simulink model "TB11_R2_FaultMod_SW"  (R2025a)
settings: Solver=FixedStepDiscrete  StartTime=0  StopTime=TB.t_end  FixedStep=TB.dt  RelTol=1e-3
InitFcn:
  | % 모델과 같은 폴더의 초기화 스크립트를 실행해 P(설계 파라미터)와 TB(시험 조건)를 만든다.
  | run(fullfile(fileparts(get_param(bdroot, 'FileName')), 'TB11_init.m'));
values from neighbouring files (symbols this model uses):
  TB = struct()    [TB11_init.m]    (also in run_TB11.m = evalin('base', 'TB'))
libraries: fl_lib x68, nesl_utility x29
(part 2 of 2)

== system TB11_R2_FaultMod_SW/StageB_Regulator/DAB_Primary/P4_leg2_low ==
  note: 스위치 셀: 이상 스위치(R_on, G_off) + 역병렬 바디 다이오드(Vf, R_d) + 출력용량 C_oss
      | 게이트: 전역 태그 "gD_P4" (> 0.5 이면 도통)
  C_oss : fl_lib/Electrical/Electrical Elements/Capacitor  c=Coss F  r=1e-6 Ohm  g=0 1/Ohm  i_specify=off  i_priority=None  i=0 A  i_nominal_specify=off  i_nominal_value=1  i_nominal_unit=A  v_specify=off  v_priority=None  v=0 V  v_nominal_specify=off  v_nominal_value=1  v_nominal_unit=V  vc_specify=off  vc_priority=High  vc=0 V  vc_nominal_specify=off  vc_nominal_value=1  vc_nominal_unit=V
  D_body : fl_lib/Electrical/Electrical Elements/Diode  Vf=Vf V  Ron=Rd Ohm  Goff=Goffd 1/Ohm  i_specify=off  i_priority=None  i=0 A  i_nominal_specify=off  i_nominal_value=1  i_nominal_unit=A  v_specify=off  v_priority=None  v=0 V  v_nominal_specify=off  v_nominal_value=1  v_nominal_unit=V
  Gate_PS : nesl_utility/Simulink-PS Converter  PhysicalDomain=network_engine_domain  SubClassName=ps_input  LeftPortType=input  RightPortType=output  PseudoPeriodic=off  Frequencies=[]  NoiseDistribution=none  NoiseParameters=[]  Unit=1  AffineConversion=off  FilteringAndDerivatives=zero  SimscapeFilterOrder=1  InputFilterTimeConstant=0.001  UdotUserProvided=0
  SW : fl_lib/Electrical/Electrical Elements/Switch  R_closed=Ron Ohm  G_open=Goff 1/Ohm  Threshold=0.5  i_specify=off  i_priority=None  i=0 A  i_nominal_specify=off  i_nominal_value=1  i_nominal_unit=A  v_specify=off  v_priority=None  v=0 V  v_nominal_specify=off  v_nominal_value=1  v_nominal_unit=V
  D : PMIOPort  Side=Left
  S : PMIOPort  Port=2  Side=Right
  wires:
  [gD_P4] -> Gate_PS/1
  connections:
  Gate_PS/RConn1 -- SW/RConn1
  SW/LConn1 -- D/RConn1 -- D_body/RConn1 -- C_oss/LConn1
  SW/RConn2 -- D_body/LConn1 -- S/RConn1 -- C_oss/RConn1

== system TB11_R2_FaultMod_SW/StageB_Regulator/DAB_Secondary/S1_leg1_high ==
  note: 스위치 셀: 이상 스위치(R_on, G_off) + 역병렬 바디 다이오드(Vf, R_d) + 출력용량 C_oss
      | 게이트: 전역 태그 "gD_S1" (> 0.5 이면 도통)
  C_oss : fl_lib/Electrical/Electrical Elements/Capacitor  c=Coss F  r=1e-6 Ohm  g=0 1/Ohm  i_specify=off  i_priority=None  i=0 A  i_nominal_specify=off  i_nominal_value=1  i_nominal_unit=A  v_specify=off  v_priority=None  v=0 V  v_nominal_specify=off  v_nominal_value=1  v_nominal_unit=V  vc_specify=off  vc_priority=High  vc=0 V  vc_nominal_specify=off  vc_nominal_value=1  vc_nominal_unit=V
  D_body : fl_lib/Electrical/Electrical Elements/Diode  Vf=Vf V  Ron=Rd Ohm  Goff=Goffd 1/Ohm  i_specify=off  i_priority=None  i=0 A  i_nominal_specify=off  i_nominal_value=1  i_nominal_unit=A  v_specify=off  v_priority=None  v=0 V  v_nominal_specify=off  v_nominal_value=1  v_nominal_unit=V
  Gate_PS : nesl_utility/Simulink-PS Converter  PhysicalDomain=network_engine_domain  SubClassName=ps_input  LeftPortType=input  RightPortType=output  PseudoPeriodic=off  Frequencies=[]  NoiseDistribution=none  NoiseParameters=[]  Unit=1  AffineConversion=off  FilteringAndDerivatives=zero  SimscapeFilterOrder=1  InputFilterTimeConstant=0.001  UdotUserProvided=0
  SW : fl_lib/Electrical/Electrical Elements/Switch  R_closed=Ron Ohm  G_open=Goff 1/Ohm  Threshold=0.5  i_specify=off  i_priority=None  i=0 A  i_nominal_specify=off  i_nominal_value=1  i_nominal_unit=A  v_specify=off  v_priority=None  v=0 V  v_nominal_specify=off  v_nominal_value=1  v_nominal_unit=V
  D : PMIOPort  Side=Left
  S : PMIOPort  Port=2  Side=Right
  wires:
  [gD_S1] -> Gate_PS/1
  connections:
  Gate_PS/RConn1 -- SW/RConn1
  SW/LConn1 -- D/RConn1 -- D_body/RConn1 -- C_oss/LConn1
  SW/RConn2 -- D_body/LConn1 -- S/RConn1 -- C_oss/RConn1

== system TB11_R2_FaultMod_SW/StageB_Regulator/DAB_Secondary/S2_leg1_low ==
  note: 스위치 셀: 이상 스위치(R_on, G_off) + 역병렬 바디 다이오드(Vf, R_d) + 출력용량 C_oss
      | 게이트: 전역 태그 "gD_S2" (> 0.5 이면 도통)
  C_oss : fl_lib/Electrical/Electrical Elements/Capacitor  c=Coss F  r=1e-6 Ohm  g=0 1/Ohm  i_specify=off  i_priority=None  i=0 A  i_nominal_specify=off  i_nominal_value=1  i_nominal_unit=A  v_specify=off  v_priority=None  v=0 V  v_nominal_specify=off  v_nominal_value=1  v_nominal_unit=V  vc_specify=off  vc_priority=High  vc=0 V  vc_nominal_specify=off  vc_nominal_value=1  vc_nominal_unit=V
  D_body : fl_lib/Electrical/Electrical Elements/Diode  Vf=Vf V  Ron=Rd Ohm  Goff=Goffd 1/Ohm  i_specify=off  i_priority=None  i=0 A  i_nominal_specify=off  i_nominal_value=1  i_nominal_unit=A  v_specify=off  v_priority=None  v=0 V  v_nominal_specify=off  v_nominal_value=1  v_nominal_unit=V
  Gate_PS : nesl_utility/Simulink-PS Converter  PhysicalDomain=network_engine_domain  SubClassName=ps_input  LeftPortType=input  RightPortType=output  PseudoPeriodic=off  Frequencies=[]  NoiseDistribution=none  NoiseParameters=[]  Unit=1  AffineConversion=off  FilteringAndDerivatives=zero  SimscapeFilterOrder=1  InputFilterTimeConstant=0.001  UdotUserProvided=0
  SW : fl_lib/Electrical/Electrical Elements/Switch  R_closed=Ron Ohm  G_open=Goff 1/Ohm  Threshold=0.5  i_specify=off  i_priority=None  i=0 A  i_nominal_specify=off  i_nominal_value=1  i_nominal_unit=A  v_specify=off  v_priority=None  v=0 V  v_nominal_specify=off  v_nominal_value=1  v_nominal_unit=V
  D : PMIOPort  Side=Left
  S : PMIOPort  Port=2  Side=Right
  wires:
  [gD_S2] -> Gate_PS/1
  connections:
  Gate_PS/RConn1 -- SW/RConn1
  SW/LConn1 -- D/RConn1 -- D_body/RConn1 -- C_oss/LConn1
  SW/RConn2 -- D_body/LConn1 -- S/RConn1 -- C_oss/RConn1

== system TB11_R2_FaultMod_SW/StageB_Regulator/DAB_Secondary/S3_leg2_high ==
  note: 스위치 셀: 이상 스위치(R_on, G_off) + 역병렬 바디 다이오드(Vf, R_d) + 출력용량 C_oss
      | 게이트: 전역 태그 "gD_S3" (> 0.5 이면 도통)
  C_oss : fl_lib/Electrical/Electrical Elements/Capacitor  c=Coss F  r=1e-6 Ohm  g=0 1/Ohm  i_specify=off  i_priority=None  i=0 A  i_nominal_specify=off  i_nominal_value=1  i_nominal_unit=A  v_specify=off  v_priority=None  v=0 V  v_nominal_specify=off  v_nominal_value=1  v_nominal_unit=V  vc_specify=off  vc_priority=High  vc=0 V  vc_nominal_specify=off  vc_nominal_value=1  vc_nominal_unit=V
  D_body : fl_lib/Electrical/Electrical Elements/Diode  Vf=Vf V  Ron=Rd Ohm  Goff=Goffd 1/Ohm  i_specify=off  i_priority=None  i=0 A  i_nominal_specify=off  i_nominal_value=1  i_nominal_unit=A  v_specify=off  v_priority=None  v=0 V  v_nominal_specify=off  v_nominal_value=1  v_nominal_unit=V
  Gate_PS : nesl_utility/Simulink-PS Converter  PhysicalDomain=network_engine_domain  SubClassName=ps_input  LeftPortType=input  RightPortType=output  PseudoPeriodic=off  Frequencies=[]  NoiseDistribution=none  NoiseParameters=[]  Unit=1  AffineConversion=off  FilteringAndDerivatives=zero  SimscapeFilterOrder=1  InputFilterTimeConstant=0.001  UdotUserProvided=0
  SW : fl_lib/Electrical/Electrical Elements/Switch  R_closed=Ron Ohm  G_open=Goff 1/Ohm  Threshold=0.5  i_specify=off  i_priority=None  i=0 A  i_nominal_specify=off  i_nominal_value=1  i_nominal_unit=A  v_specify=off  v_priority=None  v=0 V  v_nominal_specify=off  v_nominal_value=1  v_nominal_unit=V
  D : PMIOPort  Side=Left
  S : PMIOPort  Port=2  Side=Right
  wires:
  [gD_S3] -> Gate_PS/1
  connections:
  Gate_PS/RConn1 -- SW/RConn1
  SW/LConn1 -- D/RConn1 -- D_body/RConn1 -- C_oss/LConn1
  SW/RConn2 -- D_body/LConn1 -- S/RConn1 -- C_oss/RConn1

== system TB11_R2_FaultMod_SW/StageB_Regulator/DAB_Secondary/S4_leg2_low ==
  note: 스위치 셀: 이상 스위치(R_on, G_off) + 역병렬 바디 다이오드(Vf, R_d) + 출력용량 C_oss
      | 게이트: 전역 태그 "gD_S4" (> 0.5 이면 도통)
  C_oss : fl_lib/Electrical/Electrical Elements/Capacitor  c=Coss F  r=1e-6 Ohm  g=0 1/Ohm  i_specify=off  i_priority=None  i=0 A  i_nominal_specify=off  i_nominal_value=1  i_nominal_unit=A  v_specify=off  v_priority=None  v=0 V  v_nominal_specify=off  v_nominal_value=1  v_nominal_unit=V  vc_specify=off  vc_priority=High  vc=0 V  vc_nominal_specify=off  vc_nominal_value=1  vc_nominal_unit=V
  D_body : fl_lib/Electrical/Electrical Elements/Diode  Vf=Vf V  Ron=Rd Ohm  Goff=Goffd 1/Ohm  i_specify=off  i_priority=None  i=0 A  i_nominal_specify=off  i_nominal_value=1  i_nominal_unit=A  v_specify=off  v_priority=None  v=0 V  v_nominal_specify=off  v_nominal_value=1  v_nominal_unit=V
  Gate_PS : nesl_utility/Simulink-PS Converter  PhysicalDomain=network_engine_domain  SubClassName=ps_input  LeftPortType=input  RightPortType=output  PseudoPeriodic=off  Frequencies=[]  NoiseDistribution=none  NoiseParameters=[]  Unit=1  AffineConversion=off  FilteringAndDerivatives=zero  SimscapeFilterOrder=1  InputFilterTimeConstant=0.001  UdotUserProvided=0
  SW : fl_lib/Electrical/Electrical Elements/Switch  R_closed=Ron Ohm  G_open=Goff 1/Ohm  Threshold=0.5  i_specify=off  i_priority=None  i=0 A  i_nominal_specify=off  i_nominal_value=1  i_nominal_unit=A  v_specify=off  v_priority=None  v=0 V  v_nominal_specify=off  v_nominal_value=1  v_nominal_unit=V
  D : PMIOPort  Side=Left
  S : PMIOPort  Port=2  Side=Right
  wires:
  [gD_S4] -> Gate_PS/1
  connections:
  Gate_PS/RConn1 -- SW/RConn1
  SW/LConn1 -- D/RConn1 -- D_body/RConn1 -- C_oss/LConn1
  SW/RConn2 -- D_body/LConn1 -- S/RConn1 -- C_oss/RConn1

== system TB11_R2_FaultMod_SW/StageB_Regulator/HBridge/QA_high ==
  note: 스위치 셀: 이상 스위치(R_on, G_off) + 역병렬 바디 다이오드(Vf, R_d) + 출력용량 C_oss
      | 게이트: 전역 태그 "gB_AH" (> 0.5 이면 도통)
  C_oss : fl_lib/Electrical/Electrical Elements/Capacitor  c=Coss F  r=1e-6 Ohm  g=0 1/Ohm  i_specify=off  i_priority=None  i=0 A  i_nominal_specify=off  i_nominal_value=1  i_nominal_unit=A  v_specify=off  v_priority=None  v=0 V  v_nominal_specify=off  v_nominal_value=1  v_nominal_unit=V  vc_specify=off  vc_priority=High  vc=0 V  vc_nominal_specify=off  vc_nominal_value=1  vc_nominal_unit=V
  D_body : fl_lib/Electrical/Electrical Elements/Diode  Vf=Vf V  Ron=Rd Ohm  Goff=Goffd 1/Ohm  i_specify=off  i_priority=None  i=0 A  i_nominal_specify=off  i_nominal_value=1  i_nominal_unit=A  v_specify=off  v_priority=None  v=0 V  v_nominal_specify=off  v_nominal_value=1  v_nominal_unit=V
  Gate_PS : nesl_utility/Simulink-PS Converter  PhysicalDomain=network_engine_domain  SubClassName=ps_input  LeftPortType=input  RightPortType=output  PseudoPeriodic=off  Frequencies=[]  NoiseDistribution=none  NoiseParameters=[]  Unit=1  AffineConversion=off  FilteringAndDerivatives=zero  SimscapeFilterOrder=1  InputFilterTimeConstant=0.001  UdotUserProvided=0
  SW : fl_lib/Electrical/Electrical Elements/Switch  R_closed=Ron Ohm  G_open=Goff 1/Ohm  Threshold=0.5  i_specify=off  i_priority=None  i=0 A  i_nominal_specify=off  i_nominal_value=1  i_nominal_unit=A  v_specify=off  v_priority=None  v=0 V  v_nominal_specify=off  v_nominal_value=1  v_nominal_unit=V
  D : PMIOPort  Side=Left
  S : PMIOPort  Port=2  Side=Right
  wires:
  [gB_AH] -> Gate_PS/1
  connections:
  Gate_PS/RConn1 -- SW/RConn1
  SW/LConn1 -- D/RConn1 -- D_body/RConn1 -- C_oss/LConn1
  SW/RConn2 -- D_body/LConn1 -- S/RConn1 -- C_oss/RConn1

== system TB11_R2_FaultMod_SW/StageB_Regulator/HBridge/QA_low ==
  note: 스위치 셀: 이상 스위치(R_on, G_off) + 역병렬 바디 다이오드(Vf, R_d) + 출력용량 C_oss
      | 게이트: 전역 태그 "gB_AL" (> 0.5 이면 도통)
  C_oss : fl_lib/Electrical/Electrical Elements/Capacitor  c=Coss F  r=1e-6 Ohm  g=0 1/Ohm  i_specify=off  i_priority=None  i=0 A  i_nominal_specify=off  i_nominal_value=1  i_nominal_unit=A  v_specify=off  v_priority=None  v=0 V  v_nominal_specify=off  v_nominal_value=1  v_nominal_unit=V  vc_specify=off  vc_priority=High  vc=0 V  vc_nominal_specify=off  vc_nominal_value=1  vc_nominal_unit=V
  D_body : fl_lib/Electrical/Electrical Elements/Diode  Vf=Vf V  Ron=Rd Ohm  Goff=Goffd 1/Ohm  i_specify=off  i_priority=None  i=0 A  i_nominal_specify=off  i_nominal_value=1  i_nominal_unit=A  v_specify=off  v_priority=None  v=0 V  v_nominal_specify=off  v_nominal_value=1  v_nominal_unit=V
  Gate_PS : nesl_utility/Simulink-PS Converter  PhysicalDomain=network_engine_domain  SubClassName=ps_input  LeftPortType=input  RightPortType=output  PseudoPeriodic=off  Frequencies=[]  NoiseDistribution=none  NoiseParameters=[]  Unit=1  AffineConversion=off  FilteringAndDerivatives=zero  SimscapeFilterOrder=1  InputFilterTimeConstant=0.001  UdotUserProvided=0
  SW : fl_lib/Electrical/Electrical Elements/Switch  R_closed=Ron Ohm  G_open=Goff 1/Ohm  Threshold=0.5  i_specify=off  i_priority=None  i=0 A  i_nominal_specify=off  i_nominal_value=1  i_nominal_unit=A  v_specify=off  v_priority=None  v=0 V  v_nominal_specify=off  v_nominal_value=1  v_nominal_unit=V
  D : PMIOPort  Side=Left
  S : PMIOPort  Port=2  Side=Right
  wires:
  [gB_AL] -> Gate_PS/1
  connections:
  Gate_PS/RConn1 -- SW/RConn1
  SW/LConn1 -- D/RConn1 -- D_body/RConn1 -- C_oss/LConn1
  SW/RConn2 -- D_body/LConn1 -- S/RConn1 -- C_oss/RConn1

== system TB11_R2_FaultMod_SW/StageB_Regulator/HBridge/QB_high ==
  note: 스위치 셀: 이상 스위치(R_on, G_off) + 역병렬 바디 다이오드(Vf, R_d) + 출력용량 C_oss
      | 게이트: 전역 태그 "gB_BH" (> 0.5 이면 도통)
  C_oss : fl_lib/Electrical/Electrical Elements/Capacitor  c=Coss F  r=1e-6 Ohm  g=0 1/Ohm  i_specify=off  i_priority=None  i=0 A  i_nominal_specify=off  i_nominal_value=1  i_nominal_unit=A  v_specify=off  v_priority=None  v=0 V  v_nominal_specify=off  v_nominal_value=1  v_nominal_unit=V  vc_specify=off  vc_priority=High  vc=0 V  vc_nominal_specify=off  vc_nominal_value=1  vc_nominal_unit=V
  D_body : fl_lib/Electrical/Electrical Elements/Diode  Vf=Vf V  Ron=Rd Ohm  Goff=Goffd 1/Ohm  i_specify=off  i_priority=None  i=0 A  i_nominal_specify=off  i_nominal_value=1  i_nominal_unit=A  v_specify=off  v_priority=None  v=0 V  v_nominal_specify=off  v_nominal_value=1  v_nominal_unit=V
  Gate_PS : nesl_utility/Simulink-PS Converter  PhysicalDomain=network_engine_domain  SubClassName=ps_input  LeftPortType=input  RightPortType=output  PseudoPeriodic=off  Frequencies=[]  NoiseDistribution=none  NoiseParameters=[]  Unit=1  AffineConversion=off  FilteringAndDerivatives=zero  SimscapeFilterOrder=1  InputFilterTimeConstant=0.001  UdotUserProvided=0
  SW : fl_lib/Electrical/Electrical Elements/Switch  R_closed=Ron Ohm  G_open=Goff 1/Ohm  Threshold=0.5  i_specify=off  i_priority=None  i=0 A  i_nominal_specify=off  i_nominal_value=1  i_nominal_unit=A  v_specify=off  v_priority=None  v=0 V  v_nominal_specify=off  v_nominal_value=1  v_nominal_unit=V
  D : PMIOPort  Side=Left
  S : PMIOPort  Port=2  Side=Right
  wires:
  [gB_BH] -> Gate_PS/1
  connections:
  Gate_PS/RConn1 -- SW/RConn1
  SW/LConn1 -- D/RConn1 -- D_body/RConn1 -- C_oss/LConn1
  SW/RConn2 -- D_body/LConn1 -- S/RConn1 -- C_oss/RConn1

== system TB11_R2_FaultMod_SW/StageB_Regulator/HBridge/QB_low ==
  note: 스위치 셀: 이상 스위치(R_on, G_off) + 역병렬 바디 다이오드(Vf, R_d) + 출력용량 C_oss
      | 게이트: 전역 태그 "gB_BL" (> 0.5 이면 도통)
  C_oss : fl_lib/Electrical/Electrical Elements/Capacitor  c=Coss F  r=1e-6 Ohm  g=0 1/Ohm  i_specify=off  i_priority=None  i=0 A  i_nominal_specify=off  i_nominal_value=1  i_nominal_unit=A  v_specify=off  v_priority=None  v=0 V  v_nominal_specify=off  v_nominal_value=1  v_nominal_unit=V  vc_specify=off  vc_priority=High  vc=0 V  vc_nominal_specify=off  vc_nominal_value=1  vc_nominal_unit=V
  D_body : fl_lib/Electrical/Electrical Elements/Diode  Vf=Vf V  Ron=Rd Ohm  Goff=Goffd 1/Ohm  i_specify=off  i_priority=None  i=0 A  i_nominal_specify=off  i_nominal_value=1  i_nominal_unit=A  v_specify=off  v_priority=None  v=0 V  v_nominal_specify=off  v_nominal_value=1  v_nominal_unit=V
  Gate_PS : nesl_utility/Simulink-PS Converter  PhysicalDomain=network_engine_domain  SubClassName=ps_input  LeftPortType=input  RightPortType=output  PseudoPeriodic=off  Frequencies=[]  NoiseDistribution=none  NoiseParameters=[]  Unit=1  AffineConversion=off  FilteringAndDerivatives=zero  SimscapeFilterOrder=1  InputFilterTimeConstant=0.001  UdotUserProvided=0
  SW : fl_lib/Electrical/Electrical Elements/Switch  R_closed=Ron Ohm  G_open=Goff 1/Ohm  Threshold=0.5  i_specify=off  i_priority=None  i=0 A  i_nominal_specify=off  i_nominal_value=1  i_nominal_unit=A  v_specify=off  v_priority=None  v=0 V  v_nominal_specify=off  v_nominal_value=1  v_nominal_unit=V
  D : PMIOPort  Side=Left
  S : PMIOPort  Port=2  Side=Right
  wires:
  [gB_BL] -> Gate_PS/1
  connections:
  Gate_PS/RConn1 -- SW/RConn1
  SW/LConn1 -- D/RConn1 -- D_body/RConn1 -- C_oss/LConn1
  SW/RConn2 -- D_body/LConn1 -- S/RConn1 -- C_oss/RConn1

== matlab function TB11_R2_FaultMod_SW/Controller_StageB/R2_Supervisor ==
  data: t input; s output; y input; fl input; prm input; smp input
function s = prism_r2_sup_sampler(t, y, fl, prm, smp)
%#codegen
%PRISM_R2_SUP_SAMPLER  R2 보호 상태기계 표본화 실행기(TB09, MATLAB Function 블록의 진입 함수).
%
%   5 µs마다(제어기와 같은 표본 시점, 제어기보다 먼저) ctrl/prism_r2_supervisor.m을 한 번 계산하고 그 밖에는 직전 출력을 유지한다.
%   입력  t 시각, y [i_p v_s v_bus i_h v_link], fl [게이트 구동기 고장 신호, 비교기 차단 래치](한 간격 지연),
%         prm 상태기계 파라미터(TB.sup_prm), smp [dt Np]
%   출력  s 상태기계 지령 12개(prism_r2_supervisor.m 참조)

persistent sh
if isempty(sh)
    sh = zeros(12, 1);
end
k = round(t/smp(1));
if mod(k, round(smp(2))) == 0
    sh = prism_r2_supervisor(t, y, fl, prm);
end
s = sh;
end

function s = prism_r2_supervisor(t, y, fl, prm)
%#codegen
%PRISM_R2_SUPERVISOR  R2 창 조정 모듈의 측정 기반 보호 상태기계(TB09, 검증 코드 E17 r2_run의 상태기계와 같은 논리).
%
%  5 µs마다(호출 측 표본기) 측정값과 고장 신호로 운전 상태를 정하고, 제어기·게이트·바이패스·제동 저항·부하 분리 명령을 낸다.
%  상태 번호
%    0 바이패스          바이패스 닫힘, H-브리지·DAB 정지(버스 = V_A)
%    1 준비(PREP)        바이패스 + H-브리지(영벡터 또는 전류 조향: 바이패스 전류 → 0)
%    2 열림 대기         바이패스 열림, H-브리지 영벡터(또는 조향) → t_wait 뒤 제어 시작
%    3 창 조정           채택 제어기(기준 V_A → V_W 램프 뒤 V_W)
%    4 끔 램프 / 5 끔 유지(기준 = V_A 추정, |v_s| ≤ 2 V가 50 µs 이어지면) / 6 영벡터(또는 직렬전압 조향) → 바이패스
%    7 DAB 고장 유지     H-브리지는 계속 조정, DAB 정지, 링크 제동 저항으로 링크 ≤ 110 V, 400 V 부하 분리 대기
%    8 DAB 고장 램프     기준 → V_A(1 ms) → V_A 추정 추종, |v_s| ≤ 2 V가 50 µs 이어지면 → 6 → 강등
%    9 H-브리지 고장 유지  H-브리지 꺼짐(다이오드 정류), DAB 보조 루프가 링크전압으로 버스를 V_W에 붙잡음 + 제동 저항
%   10 링크 붕괴         링크 기준을 20 V/ms로 0 V까지 → 직렬전압이 다이오드 전압까지 줄어듦.
%                        링크 ≤ VL_SOFT, 또는 정체(기준 0 도달 뒤 T_STALL 동안 DV_STALL도 안 내려가고 링크 ≤ VL_STALL), 또는 T_COL_MAX → 11
%   11 소프트 바이패스   바이패스 저항을 10 Ω에서 로그 램프로 낮추되(제한 없으면 T_SOFT에 3.3 mΩ), 경로전류가 투입 시작값 + DI_SOFT를
%                        넘으면 표본마다 K_UP배로 되올린다(경로전류 조절). 3.3 mΩ에 이르거나 T_SOFT_MAX가 지나면 → 12
%   12 강등              바이패스 닫힘, Stage B 정지(버스 = V_A)
%   13 이중 고장         DAB 고장 중 H-브리지 차단: Stage A 협조 정지가 필요(이 모델 밖)
%
%  (2026-10-24 TB09 1차 결과로 추가: 회로에서는 링크 붕괴가 3.5–22 V에서 멈췄고, 남은 직렬전압을 로그 램프로 닫자 경로전류가
%   177 A까지 올랐다. 그래서 정체 감지와 경로전류 조절을 넣었다. 같은 논리를 검증 코드 E17에도 넣었다.)
%
%  (2026-10-24 TB10, 검증 코드 E20: prm이 60개면 다음을 켠다. 56개(TB09)면 이전과 같다.)
%   prm(57) 전압비 정합 유지(1): H-브리지 강등 유지(9)의 링크 기준 = (V_A − (R + R_h)i_p − 2V_D)/(n + 1), 제동 저항은 기준 추종
%   prm(58) 일시 감발(1): H-브리지 고장이면 V_A와 무관하게 400 V 부하 출력을 줄이고, V_A ≤ 상한이면 강등 T_RESTORE 뒤 되돌림
%   prm(59) 소프트 투입 시간 상한이면 주 스위치를 닫지 않고 이중 고장(13)으로
%   prm(60) T_RESTORE [s]
%   DAB 변조(EPS)와 첨두 상한은 게이트 쪽 ctrl/prism_dab_eps_map.m이 맡는다(상태 9–11, DAB 모드 1).
%
%  입력  t    시각 [s]
%        y    측정 [i_p v_s v_bus i_h v_link]
%        fl   [게이트 구동기 고장 신호(H-브리지 개방), 하드웨어 비교기 차단 래치]
%        prm  파라미터 벡터(TB09_init.m의 TB.sup_prm, 번호는 아래 코드 주석)
%  출력  s = [V_ref; 재초기화; 브리지 모드(0 제어 PWM, 1 영벡터, 2 차단, 3 조향 PWM); 조향 변조율;
%             DAB 모드(0 제어기, 1 보조 지령, 2 정지); 보조 링크전류 지령; 바이패스 소프트 저항 [Ω]; 바이패스 주 스위치(1/0);
%             제동 저항 게이트(1/0); 400 V 부하 분리(1/0); 상태 번호; 고장 검출(0 없음, 1 구동기, 2 비교기, 3 링크 창, 4 버스 창)]

persistent st t_st t_det det shed_cmd shed sw_since vb_since rv0 rv1 rt1 rtype qb amode vl0 t0 tsoft0 Rs main brk mst gsince ip_s0 stall_t stall_v ...
           curt_only restored
VW = prm(1); upper = prm(2); H = prm(3); R = prm(4); Rh = prm(5); Cs = prm(6); Lh = prm(7); itau = prm(8);
Clink = prm(9); VD = prm(10); t_ev = prm(11); ev = prm(12); pol = prm(13); prep = prm(14); cls = prm(15);
t_prep = prm(16); t_wait = prm(17); RAMP = prm(18); HOLD = prm(19); ZERO = prm(20); t_shed = prm(21);
RATE = prm(22); VL_SOFT = prm(23); T_SOFT = prm(24); R_SOFT0 = prm(25); R_ON = prm(26); T_COL_MAX = prm(27);
VL_LO = prm(28); VL_HI = prm(29); T_SW = prm(30); VB_SW = prm(31); T_VB = prm(32);
KP_B = prm(33); KI_B = prm(34); QB_MAX = prm(35); W_L = prm(36); TAU_ST = prm(37); R_OPEN = prm(38);
P_r = prm(39); link_max = prm(40); turns = prm(41); phmax = prm(42); fs = prm(43); Ldab = prm(44); vbat = prm(45);
st0 = prm(46); Ts = prm(47); VS_GATE = prm(48); T_GATE = prm(49); T_GATE_MAX = prm(50);
VL_STALL = prm(51); T_STALL = prm(52); DV_STALL = prm(53); DI_SOFT = prm(54); K_UP = prm(55); T_SOFT_MAX = prm(56);
K_DN = (R_SOFT0/R_ON)^(Ts/T_SOFT);                    % 제한에 안 걸리면 10 Ω → 3.3 mΩ를 T_SOFT에 지나는 표본당 비율
HOLD_MATCH = 0; CURTAIL = 0; SOFT_FAIL = 0; T_RESTORE = 0.5e-3;
if numel(prm) >= 60
    HOLD_MATCH = prm(57); CURTAIL = prm(58); SOFT_FAIL = prm(59); T_RESTORE = prm(60);
end

ip = y(1); vs = y(2); vb = y(3); ih = y(4); vl = y(5);
if isempty(st)
    st = st0; t_st = 0; t_det = -1; det = 0; shed_cmd = -1; shed = 0; sw_since = -1; vb_since = -1;
    rv0 = VW; rv1 = VW; rt1 = 0; rtype = 0; qb = 0; amode = 0; vl0 = 100; t0 = 0; tsoft0 = 0;
    if st0 == 3, Rs = R_OPEN; main = 0; else, Rs = R_OPEN; main = 1; end
    brk = 0; mst = 0; gsince = -1; ip_s0 = 0; stall_t = -1; stall_v = 0; curt_only = 0; restored = 0;
end
va_m = vbat/2 - R*ip;                                  % V_A 추정(배터리 전압 센서 − 경로 강하)
gwin = (st == 5 && t - t_st >= HOLD - 1e-12) || (st == 8 && t - t_st >= RAMP + HOLD - 1e-12);
if gwin && abs(vs) <= VS_GATE                          % 영벡터 진입 조건: 최소 유지 뒤 |v_s| ≤ 2 V가 50 µs 이어짐
    if gsince < 0, gsince = t; end
else
    gsince = -1;
end
gate_ok = gsince >= 0 && t - gsince >= T_GATE - 1e-12;
bridge_dead = fl(1) > 0.5 || fl(2) > 0.5;
% ---- 고장 검출 --------------------------------------------------------------------------------
if t_det < 0
    if fl(1) > 0.5, t_det = t; det = 1; end
    if fl(2) > 0.5, t_det = t; det = 2; end
    if t_det < 0 && (st == 3 || st == 4 || st == 5)
        if vl < VL_LO || vl > VL_HI
            if sw_since < 0, sw_since = t; end
            if t - sw_since >= T_SW - 1e-12, t_det = t; det = 3; end
        else
            sw_since = -1;
        end
        if abs(vb - vref_at(t, rtype, rv0, rv1, rt1, RAMP, VW, va_m)) > VB_SW
            if vb_since < 0, vb_since = t; end
            if t - vb_since >= T_VB - 1e-12, t_det = t; det = 4; end
        else
            vb_since = -1;
        end
    end
elseif fl(2) > 0.5 && det == 3 && st ~= 13 && st ~= 12 && st >= 6 && st <= 8
    st = 13; t_st = t;                                  % DAB 고장 강등 중 하드웨어 차단 → 이중 고장
end
sw_states = (st >= 1 && st <= 8);
hb_det = det == 1 || det == 2 || det == 4;
if t_det >= 0 && shed_cmd < 0 && st ~= 0 && (va_m > upper - 2 || (CURTAIL > 0.5 && hb_det))
    shed_cmd = t;
    curt_only = double(va_m <= upper - 2);              % 상한 안이면 일시 감발(강등 뒤 되돌림)
end
if shed_cmd >= 0 && t - shed_cmd >= t_shed - 1e-12 && restored < 0.5
    shed = 1;
end
if curt_only > 0.5 && st == 12 && restored < 0.5 && t - t_st >= T_RESTORE - 1e-12
    shed = 0; restored = 1;                             % 버스 = V_A ≤ 상한: 400 V 부하 출력 되돌림
end
% ---- 강등 경로 선택 ----------------------------------------------------------------------------
if (det == 1 || det == 2 || det == 4) && sw_states && st ~= 13
    if pol == 1                                          % 즉시 바이패스(비교용)
        main = 1; Rs = R_OPEN; st = 12; t_st = t;
    elseif pol == 2                                      % 바로 붕괴(비교용)
        amode = 1; t0 = t; vl0 = vl; st = 10; t_st = t;
    else
        st = 9; t_st = t; amode = 0; qb = 0;
    end
elseif det == 3 && (st == 3 || st == 4 || st == 5)
    if pol == 2 && shed_cmd >= 0                         % 제동 저항으로 유지
        st = 7; t_st = t;
    else
        rv0 = vref_at(t, rtype, rv0, rv1, rt1, RAMP, VW, va_m); rv1 = va_m; rt1 = t; rtype = 1; st = 8; t_st = t;
    end
end
% ---- 링크 붕괴 정체 감지(기준이 0에 닿은 뒤) ------------------------------------------------------------
stalled = false;
if st == 10 && t - t_st >= vl0/RATE - 1e-12
    if stall_t < 0 || stall_v - vl >= DV_STALL
        stall_t = t; stall_v = vl;
    end
    stalled = (t - stall_t >= T_STALL - 1e-12) && vl <= VL_STALL;
end
% ---- 정상 순서와 강등 진행 --------------------------------------------------------------------------
if st == 0 && ev == 1 && t >= t_ev && vbat/2 >= VW + H
    st = 1; t_st = t;
elseif st == 1 && t - t_st >= t_prep - 1e-12
    main = 0; Rs = R_OPEN; st = 2; t_st = t;
elseif st == 2 && t - t_st >= t_wait - 1e-12
    rv0 = va_m; rv1 = VW; rt1 = t; rtype = 1; st = 3; t_st = t;
elseif st == 3 && ev == 2 && t >= t_ev && t_det < 0 && vbat/2 <= VW - H
    rv0 = vref_at(t, rtype, rv0, rv1, rt1, RAMP, VW, va_m); rv1 = va_m; rt1 = t; rtype = 1; st = 4; t_st = t;
elseif st == 4 && t - t_st >= RAMP - 1e-12
    rtype = 2; st = 5; t_st = t;                         % 램프 뒤에는 기준이 V_A 추정을 따라간다
elseif st == 5 && t - t_st >= HOLD - 1e-12 && (gate_ok || t - t_st >= T_GATE_MAX - 1e-12)
    st = 6; t_st = t;
elseif st == 7 && shed > 0.5
    rv0 = vref_at(t, rtype, rv0, rv1, rt1, RAMP, VW, va_m); rv1 = va_m; rt1 = t; rtype = 1; st = 8; t_st = t;
elseif st == 8 && t - t_st >= RAMP - 1e-12 && rtype ~= 2
    rtype = 2;
elseif st == 8 && t - t_st >= RAMP + HOLD - 1e-12 && (gate_ok || t - t_st >= RAMP + T_GATE_MAX - 1e-12)
    st = 6; t_st = t;
elseif st == 6 && t - t_st >= ZERO - 1e-12
    main = 1; Rs = R_OPEN;
    if t_det >= 0, st = 12; else, st = 0; end
    t_st = t;
elseif st == 9 && (shed_cmd < 0 || shed > 0.5)
    amode = 1; t0 = t; vl0 = vl; st = 10; t_st = t;
elseif st == 10 && (vl <= VL_SOFT || stalled || t - t_st >= T_COL_MAX - 1e-12)
    if pol == 5
        main = 1; Rs = R_OPEN; st = 12;
    else
        tsoft0 = t; ip_s0 = ip; Rs = R_SOFT0; st = 11;
    end
    t_st = t;
elseif st == 11 && (Rs <= R_ON*(1 + 1e-9) || t - t_st >= T_SOFT_MAX - 1e-12)
    if Rs > R_ON*(1 + 1e-9) && SOFT_FAIL > 0.5
        st = 13; t_st = t;                              % 시간 상한: 닫지 않고 이중 고장(Stage A 협조 정지)
    else
        main = 1; Rs = R_OPEN; st = 12; t_st = t;
    end
end
if st == 11 && t > tsoft0 + 1e-12                        % 소프트 투입(경로전류 조절)
    if ip > ip_s0 + DI_SOFT
        Rs = min(Rs*K_UP, R_SOFT0);
    else
        Rs = max(Rs/K_DN, R_ON);
    end
end
% ---- 지령 --------------------------------------------------------------------------------------
vref = vref_at(t, rtype, rv0, rv1, rt1, RAMP, VW, va_m);
rst = double(st == 0 || st == 1 || st == 2 || st == 6 || st >= 9);
steer = (st == 1 || st == 2) && prep > 0.5 || (st == 6 && cls > 0.5);
if st == 3 || st == 4 || st == 5 || st == 7 || st == 8
    bmode = 0;
elseif steer
    bmode = 3;
elseif st == 1 || st == 2 || st == 6
    bmode = 1;
else
    bmode = 2;
end
if bridge_dead, bmode = 2; end
if steer
    if st == 6, ihs = ip - Cs*vs/TAU_ST; else, ihs = ip; end
    mst = min(max((vs + Rh*ih + Lh/itau*(ihs - ih))/max(vl, 1), -0.95), 0.95);
end
% 보조 링크 루프(H-브리지 강등 9–11)
icmd_aux = 0; vlr = vl;
if st >= 9 && st <= 11
    if amode == 0 && HOLD_MATCH > 0.5
        vlr = min(max((vbat/2 - (R + Rh)*ip - 2*VD)/(turns + 1), 0), 100);   % DAB 전압비 정합(n·v_link = v_bus)
    elseif amode == 0
        e = vb - VW;
        qb = min(max(qb + Ts*KI_B*e, -QB_MAX), QB_MAX);
        ff = vbat/2 - (R + Rh)*ip - 2*VD - VW;
        vlr = min(max(ff + KP_B*e + qb, 0), 110);
    else
        vlr = max(vl0 - RATE*(t - t0), 0);
    end
    sps = max(vb, 0)*turns*phmax*(1 - phmax/pi)/(2*pi*fs*Ldab);
    lim = min([link_max, sps, P_r/max(vl, 1e-3)]);
    icmd_aux = min(max(-abs(ih) + Clink*W_L*(vlr - vl), -lim), lim);
end
if st >= 9 && st <= 11
    dmode = 1;
elseif st == 3 || st == 4 || st == 5 || st == 7 || st == 8
    dmode = 0;
else
    dmode = 2;
end
if det == 3, dmode = 2; end                              % DAB 고장: DAB 게이트는 고장 주입으로 이미 꺼져 있음
% 제동 저항(정책 4·5, DAB 정책 2). H-브리지 강등 유지(9) 중에는 링크 과전압 보호만(110 V), 붕괴·소프트 투입(10·11) 중에는
% 링크 기준 + 5 V 위에서 켠다(2026-10-24: 유지 중 기준 추종 제동은 경로전류 첨두를 키워 E17에서 W410 103 A로 불통과)
if (pol == 4 || pol == 5) && st == 9 && HOLD_MATCH < 0.5
    if vl > 110, brk = 1; elseif vl < 105, brk = 0; end
elseif (pol == 4 || pol == 5) && st == 9
    if vl > vlr + 5, brk = 1; elseif vl < vlr + 2, brk = 0; end   % 정합 유지: DAB 정격 밖 전력을 제동 저항이
elseif (pol == 4 || pol == 5) && st >= 10 && st <= 11
    if vl > vlr + 5, brk = 1; elseif vl < vlr + 2, brk = 0; end
elseif pol == 2 && det == 3 && (st == 7 || st == 8 || st == 6)
    if vl > 110, brk = 1; elseif vl < 105, brk = 0; end
else
    brk = 0;
end
s = [vref; rst; bmode; mst; dmode; icmd_aux; Rs; main; brk; shed; st; det];
end

function v = vref_at(t, rtype, v0, v1, t1, RAMP, VW, va_m)
% 기준전압: 0 = V_W, 1 = v0 → v1 직선 램프(RAMP), 2 = V_A 추정 추종(끔·DAB 고장 램프 뒤)
if rtype < 0.5
    v = VW;
elseif rtype < 1.5
    v = v0 + (v1 - v0)*min((t - t1)/RAMP, 1);
else
    v = va_m;
end
end

== matlab function TB11_R2_FaultMod_SW/DAB_Loss_Model/DAB_Loss ==
  data: t input; iloss output; vl input; il input; iL input; vb input; prm input; ploss0 input
function iloss = prism_dab_loss(t, vl, il, iL, vb, prm, ploss0)
%#codegen
%PRISM_DAB_LOSS  DAB 손실 등가 전류(검증 모델과 같은 손실 모델).
%
%   스위칭 회로의 DAB에는 권선저항 R_dab만 있고 스위칭·자기 손실이 없다. 검증 모델(E12)은 평균모델과 같은
%   방향별 효율 η = 0.96을 쓰기 위해, 직전 제어주기의 평균 링크전력 p̄로 정한 손실
%       P_loss = (1/η − 1)·max(p̄, 0) + (1 − η)·max(−p̄, 0) − R_dab·mean(i_L²)   (0 이상)
%   을 버스에서 끄는 전류 P_loss/v_bus로 넣는다. 이 블록은 같은 계산을 해서 버스의 제어 전류원에 준다.
%   이렇게 하면 정상상태의 DAB 총손실이 검증 모델과 같아, 두 모델의 차이는 스위칭 동작에서만 나온다.
%
%   입력  t 시각, vl 링크전압, il 링크 직류전류(2차 브리지 → 링크), iL 누설 전류, vb 버스전압
%         prm [dt Np η R_dab]   ploss0 초기 손실 [W](평형점 링크전력 기준)
%   출력  iloss  버스에서 끄는 손실 전류 [A]

persistent accP accI2 ploss started
if isempty(started)
    started = 1; accP = 0; accI2 = 0; ploss = ploss0;
end
dt = prm(1); Np = round(prm(2)); eta = prm(3); Rd = prm(4);
k = round(t/dt);
accP = accP + vl*il;
accI2 = accI2 + iL*iL;
if mod(k, Np) == Np - 1                       % 주기 마지막 간격에서 갱신(다음 주기에 적용)
    pbar = accP/Np;
    lossEta = (1/eta - 1)*max(pbar, 0) + (1 - eta)*max(-pbar, 0);
    ploss = max(lossEta - Rd*accI2/Np, 0);
    accP = 0; accI2 = 0;
end
iloss = ploss/max(vb, 1);
end

== matlab function TB11_R2_FaultMod_SW/Controller_StageB/Adopted_Controller ==
  data: t input; u output; y input; prm input; init input; tab input; smp input; dg output
function [u, dg] = prism_ctrl_sampler_r2b(t, y, prm, init, tab, smp)
%#codegen
%PRISM_CTRL_SAMPLER_R2B  채택 제어기 표본화 실행기의 R2 보호 상태기계판(TB09, MATLAB Function 블록의 진입 함수).
%
%   ctrl/prism_ctrl_sampler_r2.m과 같이 5 µs마다 제어기를 한 번 계산하고, 상태기계(ctrl/prism_r2_supervisor.m)의
%   지령을 함께 받는다.
%     y(10) V_ref, y(11) 재초기화, y(12) 브리지 모드(3이면 상태기계의 조향 변조율을 PWM 비교값으로),
%     y(13) 조향 변조율, y(14) DAB 모드(1이면 보조 링크전류 지령), y(15) 보조 링크전류 지령
%   제어 법칙은 prism_stageB_controller.m 그대로다(보조 지령은 링크전압 PI 대신 들어간다).
%
%   입력  y = [i_p v_s v_bus i_h v_link V_bat i_link_avg φ_c0 φ_c1 | 상태기계 지령 6개]
%   출력  u, dg : ctrl/prism_ctrl_sampler.m과 같음

persistent uh dgh
if isempty(uh)
    uh = [init(3); 0];
    dgh = zeros(6, 1);
end
k = round(t/smp(1));
if mod(k, round(smp(2))) == 0
    prm2 = prm;
    prm2(9) = y(10);                                   % 시변 버스 기준전압
    [uh, dgh] = prism_stageB_controller(y(1:9), prm2, init, tab, y(11), [double(y(14) == 1); y(15)]);
    if round(y(12)) == 3
        uh(1) = y(13);                                 % 전류 조향: 상태기계가 정한 변조율
    end
end
u = uh;
dg = dgh;
end

function [u, dg] = prism_stageB_controller(y, prm, init, tab, rst, aux)
%#codegen
%PRISM_STAGEB_CONTROLLER  Stage B 채택 제어기 1회 계산(제어주기 5 µs, 반송파 최댓값에서 표본).
%
%  검증 코드(model_stage_b_switching.run_core의 제어 부분)와 같은 법칙이다.
%   (1) 1주기 예측: 고속 상태 [i_p, v_s, i_h]를 직전 변조율로 5 µs 앞까지 공칭 모델로 적분(중점법 5단계)
%   (2) 상태궤환 + 버스전압 적분 → 브리지 전류지령(±84 A 포화, 역포화 보정)
%   (3) 내부 전류 법칙 → 변조율 m(±0.95)
%   (4) 링크전압 PI + 소비전류 앞먹임 → DAB 링크전류 지령(정격 80 A·8 kW·SPS 한계)
%   (5) DAB 링크전류 → 위상: 누설 인덕턴스 −10 % 기준 앞먹임 + 측정 전류비 ρ̂ 보정 + 저전류 가산 보정 ε̂
%   (6) H-브리지 데드타임 보상: 교정표 × 전류 스케줄 κ(20 A 이하 0.6 → 80 A 1.0)
%
%  입력
%   y    = [i_p v_s v_bus i_h v_link V_bat i_link_avg ph_c0 ph_c1]  (표본값)
%          i_link_avg : 직전 제어주기의 DAB 링크 직류전류 평균(측정)
%          ph_c0/ph_c1: 그 주기의 두 반주기 중심에서 적용된 유효 위상(게이트 생성기가 기록)
%   prm  = 상수 벡터(prism_hub_params의 P.ctrl_prm)
%           1 L  2 Cs  3 Cb  4 R  5 Lh  6 Rh  7 Clink  8 Ts  9 vref  10 vlink  11 mmax  12 refmax
%          13 link_max  14 power_max  15 link_bw  16 inner_tau  17 Ldab  18 fs  19 turns  20 phmax
%          21–25 K  26 lmin(0.9)  27 ρ̂ 이득  28 ρ̂ 최소 전류  29 ε̂ 이득  30 ε̂ 상한
%          31 κ 경부하 비율  32 κ 시작 전류  33 κ 1 도달 전류  34 교정표 기준 링크전압  35 예측 단계 수
%          36 예측 사용(1)  37 데드타임 보상 사용(1)
%   init = [q0 q_link0 m0 i_link0]   (평형점에서 시작: 적분기가 지령 = i_p가 되도록)
%   tab  = [i_grid; E(i)]            데드타임 교정표(전류별 상승 전이 한 번의 전압·시간 손실)
%   rst  = (선택, R2 창 조정 모듈 TB08) 1이면 이번 표본에서 무충격 재초기화한다. 적분기를 지령 = 경로전류가 되도록 맞추고
%          링크 적분기·직전 변조율·ρ̂·ε̂를 처음 값(0, 0, 1, 0)으로 둔다(검증 코드 StageBController.reset과 같은 계산).
%          영벡터·바이패스로 제어 출력이 쓰이지 않는 동안 매 표본 다시 맞춰, 제어를 시작할 때 충격이 없게 한다.
%          네 입력으로 부르면(TB04–TB07) 이 기능은 없고 계산은 이전과 같다.
%   aux  = (선택, R2 보호 상태기계 TB09) [보조 지령 사용(1/0); 보조 링크전류 지령 A]. 1이면 링크전압 PI 대신 보조 지령을
%          DAB 링크전류 지령으로 쓴다(H-브리지 차단 강등에서 상태기계의 보조 루프가 링크전압으로 버스를 붙잡을 때).
%          위상 계산(전류비·저전류 보정 포함)은 같다. 다섯 입력 이하로 부르면 이전과 같다.
%  출력
%   u  = [PWM 비교값(데드타임 보상 후); DAB 유효 위상 지령 rad]
%   dg = [m 지령(보상 전); 링크전류 지령; 브리지 전류지령; ρ̂; ε̂; 예측 링크전류]

persistent q qlink mprev rho epsA vbprev started
if isempty(started)
    q = init(1); qlink = init(2); mprev = init(3); rho = 1; epsA = 0; vbprev = y(3); started = 1;
end

L = prm(1); Cs = prm(2); R = prm(4); Lh = prm(5); Rh = prm(6); Clink = prm(7); Ts = prm(8);
vref = prm(9); vlink = prm(10); mmax = prm(11); refmax = prm(12);
link_max = prm(13); power_max = prm(14); link_bw = prm(15); itau = prm(16);
Ldab = prm(17); fs = prm(18); turns = prm(19); phmax = prm(20);
K = prm(21:25);
lmin = prm(26); est_g = prm(27); est_min = prm(28); eps_g = prm(29); eps_max = prm(30);
k_scale = prm(31); k_from = prm(32); k_full = prm(33); Vtab = prm(34); nsub = prm(35);

ip = y(1); vs = y(2); vb = y(3); ih = y(4); vl = y(5); vbat = y(6);
il_meas = y(7); ph_c0 = y(8); ph_c1 = y(9);
if nargin >= 5                                   % (R2, TB08) 무충격 재초기화
    if rst > 0.5
        q = -(ip + K(1)*ip + K(2)*vs + K(3)*vb + K(4)*ih)/K(5);
        qlink = 0; mprev = 0; rho = 1; epsA = 0; vbprev = vb;
    end
end

% ---- (1) 1주기 예측 -----------------------------------------------------------------
sip = ip; svs = vs; sih = ih;
if prm(36) > 0.5
    m = mprev; h = Ts/nsub;
    for s = 1:nsub
        a1 = (vbat/2 - R*sip + svs - vb)/L;
        a2 = (sih - sip)/Cs;
        a3 = (m*vl - svs - Rh*sih)/Lh;
        mp = sip + 0.5*h*a1;  mv = svs + 0.5*h*a2;  mh = sih + 0.5*h*a3;
        b1 = (vbat/2 - R*mp + mv - vb)/L;
        b2 = (mh - mp)/Cs;
        b3 = (m*vl - mv - Rh*mh)/Lh;
        sip = sip + h*b1;  svs = svs + h*b2;  sih = sih + h*b3;
    end
end
% ---- (2) 상태궤환 + 적분 -----------------------------------------------------------
raw  = -(K(1)*sip + K(2)*svs + K(3)*vb + K(4)*sih) - K(5)*q;
iref = min(refmax, max(-refmax, raw));
q = q + Ts*(vref - vb) + 0.1*(iref - raw)/(-K(5));
% ---- (3) 내부 전류 법칙 → 변조율 ---------------------------------------------------
vlx = max(vl, 1);                                % (보상 계산용 하한)
mraw = (svs + Rh*sih + Lh/itau*(iref - sih))/vl;
mcmd = min(mmax, max(-mmax, mraw));
% ---- (4) 링크전압 PI + 앞먹임 → DAB 링크전류 지령 ---------------------------------
w = 2*pi*link_bw;
rawlink = mcmd*sih + Clink*(2*0.7*w*(vlink - vl) + w*w*qlink);
sps = max(vb, 0)*turns*phmax*(1 - phmax/pi)/(2*pi*fs*Ldab);
lim = min(min(link_max, sps), power_max/max(vl, 1e-9));
icmd = min(lim, max(-lim, rawlink));
qlink = qlink + Ts*(vlink - vl) + 0.1*(icmd - rawlink)/(Clink*w*w);
if nargin >= 6                                   % (R2 보호, TB09) 보조 링크전류 지령
    if aux(1) > 0.5
        icmd = aux(2); qlink = 0;
    end
end
mprev = mcmd;
% ---- (5) DAB 전류비·저전류 보정 → 위상 ----------------------------------------------
% 직전 주기 두 반주기 중심에 적용된 위상의 예측 전류. 그 위상을 적용할 때 쓰인 버스전압은 직전 표본값이다
% (검증 모델: 반주기 중심에서 그때의 측정 버스전압으로 예측 전류를 계산).
il_pred = 0.5*(ipred(ph_c0, vbprev, turns, fs, Ldab, lmin) + ipred(ph_c1, vbprev, turns, fs, Ldab, lmin));
vbprev = vb;
dph = abs(ph_c1 - ph_c0);
if abs(il_pred) >= est_min && il_meas*il_pred > 0 && dph < 0.035
    rho = rho + est_g*(il_meas/il_pred - rho);
    rho = min(max(rho, 0.75), 1.25);
end
if eps_g > 0
    if abs(il_pred) < est_min && dph < 0.035
        epsA = epsA + eps_g*((il_meas - rho*il_pred) - epsA);
    elseif abs(il_pred) >= est_min
        epsA = epsA - eps_g*epsA;
    end
    epsA = min(max(epsA, -eps_max), eps_max);
end
ph_new = phase_ff((icmd - epsA)/rho, vb, turns, fs, Ldab, lmin, phmax);
% ---- (6) H-브리지 데드타임 보상 ----------------------------------------------------
m_pwm = mcmd;
if prm(37) > 0.5
    kap = k_scale + (1 - k_scale)*min(max((abs(sih) - k_from)/max(k_full - k_from, 1e-9), 0), 1);
    m_pwm = mcmd - kap*dt_error_tab(mcmd, sih, vlx, Lh, fs, tab, Vtab)/vlx;
end
u  = [m_pwm; ph_new];
dg = [mcmd; icmd; iref; rho; epsA; il_pred];
end

% ======================================================================================
function i = ipred(ph, vb, turns, fs, Ldab, lb)
% 위상 ph에서 SPS 식이 주는 링크전류(누설 인덕턴스 = 공칭의 lb배 가정)
k = turns*max(vb, 1)/(2*pi*fs*Ldab*lb);
i = k*ph*(1 - abs(ph)/pi);
end

function ph = phase_ff(il, vb, turns, fs, Ldab, lb, phmax)
% 링크전류 → SPS 위상 앞먹임(|φ| ≤ φ_max)
k = turns*max(vb, 1)/(2*pi*fs*Ldab*lb);
a = min(abs(il)/(pi*k/4), 1);
ph = min(pi/2*(1 - sqrt(1 - a)), phmax);
if il < 0, ph = -ph; end
end

function d = dt_error_tab(m, i, V, Lh, f, tab, Vtab)
% 유니폴라 PWM 한 주기의 브리지 평균 전압오차 [V]: 리플 극값 전류에서의 전이별 손실을 교정표에서 읽는다.
sg = 1;
if m < 0, m = -m; i = -i; sg = -1; end
r = V*m*(1 - m)/(4*Lh*f);
imin = i - r; imax = i + r;
d = sg*2*(tab_interp(-imax, tab) - tab_interp(imin, tab))*(V/Vtab)*f;
end

function e = tab_interp(x, tab)
% 선형 보간(범위 밖은 끝값) — numpy.interp와 같음
n = size(tab, 2);
if x <= tab(1, 1), e = tab(2, 1); return; end
if x >= tab(1, n), e = tab(2, n); return; end
lo = 1; hi = n;
while hi - lo > 1
    mid = floor((lo + hi)/2);
    if tab(1, mid) <= x, lo = mid; else, hi = mid; end
end
w = (x - tab(1, lo))/(tab(1, hi) - tab(1, lo));
e = tab(2, lo) + w*(tab(2, hi) - tab(2, lo));
end

== matlab function TB11_R2_FaultMod_SW/Gate_StageB/StageB_Gate ==
  data: t input; g output; uc input; ilink input; prm input; init input; eps input; aux output
function [g, aux] = prism_gate_stageB_e(t, uc, ilink, prm, init, eps)
%#codegen
%PRISM_GATE_STAGEB_E  Stage B 게이트 생성기 + DAB 고장 모드 변조(EPS, TB10). eps(1) = 0이면 ctrl/prism_gate_stageB.m과 같다.
%
%  EPS(1차 내부 위상천이): SPS 생성기가 정한 1차 에지(가상 에지)에서 레그 1(P1·P2)은 그대로 바꾸고, 레그 2(P3·P4)는
%  D1·T/2 늦게 바꾼다. 1차 전압은 −V → 0(레그 1만 바뀜) → +V(레그 2도 바뀜)가 되어 반주기마다 (1 − D1)·T/2 폭의 펄스가 된다.
%  D1은 상향 가상 에지에서 잡아 그 주기의 하향 에지까지 그대로 쓴다(양·음 펄스 폭이 같아 1차 직류 편류가 생기지 않는다).
%  위상은 eps(2)를 SPS 위상 지령 대신 쓰므로, 위상 변화의 직류 편류 방지(전이 반주기 평균)는 SPS와 같이 적용된다.
%  위상 기준: 2차 상향 에지 − 가상 에지 = φ, 1차 펄스 시작 = 가상 에지 + D1·T/2(검증 코드 dab_modulation.eps_params와 같은 정의).
%
%  추가 입력  eps  [EPS 켬(1/0); 위상 φ [rad]; 내부 위상비 D1(0–0.95)]  (ctrl/prism_dab_eps_map.m)
%
%  아래는 SPS 생성기 설명(그대로):
%PRISM_GATE_STAGEB  Stage B 게이트 생성기(적분 간격 dt = 5 ns마다 실행).
%
%  H-브리지 : 유니폴라 PWM. 삼각 반송파 c(t)는 제어주기 시작(표본 시점)에서 +1, 반주기에서 −1.
%             레그 A 상측 목표 = (m > c), 레그 B 상측 목표 = (−m > c). 목표가 바뀌면 두 소자를 데드타임 동안
%             끄고(출력용량 충방전·다이오드 도통은 회로가 정함) 새 소자를 켠다.
%  DAB      : 50 % 구형파 두 풀브리지, 단일 위상천이. 에지는 반송파 반주기 중심 c_j에 대칭(1차 c_j − δ/2,
%             2차 c_j + δ/2, δ = φ·T/2π)으로 놓고, 지령은 도착 후 첫 반주기 중심에서 반영한다.
%             전이 반주기의 위상차를 이전·새 위상의 평균으로 두는 갱신(A ← −A + 2Δ, Δ = (A + δ_new)/2)으로
%             위상이 바뀔 때 변압기 직류 편류가 생기지 않게 한다(검증 코드와 같은 알고리즘).
%             에지 시각은 dt 격자에 반올림하고, 실제 실행 시각으로 다음 반주기의 A를 계산한다.
%  링크전류 : DAB 2차 브리지가 링크로 보내는 직류전류를 제어주기마다 평균해 다음 표본에 넘긴다.
%
%  입력  t      시뮬레이션 시각(Digital Clock, dt 간격)
%        uc     [PWM 비교값; DAB 유효 위상 rad]  (제어기 출력, 전달지연 뒤)
%        ilink  DAB 2차 브리지 → 링크 직류전류 [A](순시)
%        prm    [dt Np td_h(간격 수) td_d(간격 수) T]
%        init   [PWM 비교값 초기값, 위상 초기값, 링크전류 초기값]
%  출력  g      [A상측 A하측 B상측 B하측 | P1 P2 P3 P4 | S1 S2 S3 S4]  (1 = 켬)
%               DAB 브리지: 상태 +1 → 1·4번 켬, −1 → 2·3번 켬(1·2번이 레그 1, 3·4번이 레그 2, 홀수 = 상측)
%        aux    [링크전류 주기 평균; 그 주기 두 반주기 중심의 위상 φ_c0, φ_c1; 반송파; 1차 상태; 2차 상태]

persistent started kA kB tgtA tgtB A ph_tgt p_t s_t p_h s_h p_j s_j p_state s_state p_te s_te ...
           acc il_avg phc0 phc1 lat0 lat1 D1c l2_t l2_tgt l2_hi l2_te l2_pend
dt = prm(1); Np = prm(2); ndh = prm(3); ndd = prm(4); T = prm(5);
Nh = round(Np/2);
k  = round(t/dt);                     % 적분 간격 번호(0부터)
t0 = k*dt;

if isempty(started)
    started = 1;
    m0 = init(1); ph0 = init(2);
    c0 = 1;                            % k = 0의 반송파
    tgtA = double(m0 > c0); tgtB = double(-m0 > c0);
    kA = -1e9; kB = -1e9;              % 데드타임 없이 시작
    ph_tgt = ph0;
    d0 = ph0/(2*pi)*T;
    A = d0;
    p_t = [1e30 1e30]; s_t = [1e30 1e30]; p_h = [0 0]; s_h = [0 0];
    p_te = -1; s_te = -1;
    if d0 > 0
        p_j = 1; p_h(1) = -d0/2; p_state = 1;  s_j = 0; s_state = -1;
    elseif d0 < 0
        s_j = 1; s_h(1) = d0/2;  s_state = 1;  p_j = 0; p_state = -1;
    else
        p_j = 0; s_j = 0; p_state = -1; s_state = -1;
    end
    acc = 0; il_avg = init(3); phc0 = ph0; phc1 = ph0; lat0 = ph0; lat1 = ph0;
    D1c = 0; l2_t = 1e30; l2_tgt = double(p_state < 0); l2_hi = l2_tgt; l2_te = -1; l2_pend = 0;
end

m = uc(1);
if eps(1) > 0.5
    ph_tgt = eps(2);                  % 고장 모드 변조: 상태기계 쪽 EPS 지령의 위상
else
    ph_tgt = uc(2);
end

% ---------------- H-브리지 유니폴라 PWM -------------------------------------------------
kin = mod(k, Np);
c = 4*abs(kin/Np - 0.5) - 1;
nA = double(m > c); nB = double(-m > c);
if nA ~= tgtA, tgtA = nA; kA = k; end
if nB ~= tgtB, tgtB = nB; kB = k; end
okA = (k - kA) >= ndh; okB = (k - kB) >= ndh;
gA_hi = double(okA && tgtA == 1); gA_lo = double(okA && tgtA == 0);
gB_hi = double(okB && tgtB == 1); gB_lo = double(okB && tgtB == 0);

% ---------------- DAB 위상 갱신(반주기 중심) --------------------------------------------
if mod(k, Nh) == 0
    j = k/Nh; cj = t0;
    if j >= 1
        jm = mod(j - 1, 2) + 1;
        A = -A + 2*(s_h(jm) - p_h(jm));
    end
    dtg = ph_tgt/(2*pi)*T;
    D = 0.5*(A + dtg);
    jj = mod(j, 2) + 1;
    p_done = p_j > j; s_done = s_j > j;
    if p_done && ~s_done
        s_t(jj) = max(cj, p_h(jj) + D);
    elseif s_done && ~p_done
        p_t(jj) = max(cj, s_h(jj) - D);
    elseif ~p_done && ~s_done
        if D >= 0
            p_t(jj) = cj; s_t(jj) = cj + D;
        else
            s_t(jj) = cj; p_t(jj) = cj - D;
        end
    end
    if p_done, tpj = p_h(jj); else, tpj = p_t(jj); end
    if s_done, tsj = s_h(jj); else, tsj = s_t(jj); end
    D1 = 0.5*(-A + 2*(tsj - tpj) + dtg);
    cn = (j + 1)*Nh*dt;
    p_t(3 - jj) = cn - D1/2; s_t(3 - jj) = cn + D1/2;
    if mod(j, 2) == 0, phc0 = ph_tgt; else, phc1 = ph_tgt; end
end
% ---------------- DAB 에지 실행(가장 가까운 간격에 반올림) ------------------------------
sp = mod(p_j, 2) + 1;
if p_t(sp) < t0 + 0.5*dt
    if mod(p_j, 2) == 0
        p_state = 1;
        if eps(1) > 0.5, D1c = min(max(eps(3), 0), 0.95); else, D1c = 0; end   % 상향 에지에서 D1을 잡는다
    else
        p_state = -1;
    end
    p_te = t0; p_h(sp) = t0; p_t(sp) = 1e30; p_j = p_j + 1;
    if l2_pend > 0.5                   % (위상 전이로 반주기가 짧아진 경우) 남은 레그 2 전환을 먼저 끝낸다
        l2_hi = l2_tgt; l2_te = t0; l2_pend = 0;
    end
    l2_tgt = double(p_state < 0); l2_t = t0 + D1c*T/2; l2_pend = 1;   % 레그 2: −1 상태에서 상측(P3) 켬
end
if l2_pend > 0.5 && l2_t < t0 + 0.5*dt
    l2_hi = l2_tgt; l2_te = t0; l2_pend = 0;
end
ss = mod(s_j, 2) + 1;
if s_t(ss) < t0 + 0.5*dt
    if mod(s_j, 2) == 0, s_state = 1; else, s_state = -1; end
    s_te = t0; s_h(ss) = t0; s_t(ss) = 1e30; s_j = s_j + 1;
end
p_ok = (t0 - p_te) >= ndd*dt - 0.5*dt;
s_ok = (t0 - s_te) >= ndd*dt - 0.5*dt;
gP = [0 0 0 0]; gS = [0 0 0 0];
if p_ok                                % 레그 1(P1 상측, P2 하측)
    if p_state > 0, gP(1:2) = [1 0]; else, gP(1:2) = [0 1]; end
end
if (t0 - l2_te) >= ndd*dt - 0.5*dt     % 레그 2(P3 상측, P4 하측), 자기 전환 뒤 데드타임
    if l2_hi > 0.5, gP(3:4) = [1 0]; else, gP(3:4) = [0 1]; end
end
if s_ok
    if s_state > 0, gS = [1 0 0 1]; else, gS = [0 1 1 0]; end
end

% ---------------- 링크전류 주기 평균(표본 직전 간격에서 확정) -------------------------
acc = acc + ilink;
if kin == Np - 1
    il_avg = acc/Np; acc = 0;
    lat0 = phc0; lat1 = phc1;
end

g = [gA_hi gA_lo gB_hi gB_lo gP gS]';
aux = [il_avg; lat0; lat1; c; p_state; s_state];
end

== matlab function TB11_R2_FaultMod_SW/Gate_StageB/R2_Gate_Protect ==
  data: t input; gb output; g input; sup input; meas input; prm input; fl output
function [gb, fl] = prism_r2_gate_b(t, g, sup, meas, prm)
%#codegen
%PRISM_R2_GATE_B  R2 보호 상태기계의 게이트 재정의(TB09, 적분 간격마다 실행): 하드웨어 비교기, 고장 주입, 모드별 게이트.
%
%  입력  g     게이트 생성기 출력 [A상측 A하측 B상측 B하측 | P1–P4 | S1–S4] (ctrl/prism_gate_stageB.m)
%        sup   상태기계 지령 [브리지 모드(0 제어 PWM, 1 영벡터, 2 차단, 3 조향 PWM); DAB 모드(0 제어기, 1 보조, 2 정지);
%              바이패스 주 스위치; 제동 저항 게이트; 상태 번호]
%        meas  [i_p i_h v_link v_s v_bus]
%        prm   [dt T_HW I_HW VL_HW VS_HW 상한 고장종류(0 없음, 1 H-브리지 개방, 2 DAB 정지) 고장시각 T_GDF]
%  출력  gb    [H-브리지 4 | DAB 8 | 바이패스 주 스위치 | 제동 저항]
%        fl    [게이트 구동기 고장 신호(H-브리지 개방, T_GDF 뒤); 하드웨어 비교기 차단 래치]
%  하드웨어 비교기는 H-브리지가 동작하는 동안(차단·고장 전) 연속 감시한다: |i_p|·|i_h| > I_HW, v_link > VL_HW,
%  |v_s| > VS_HW, 그리고 정상 조정 상태(1–5)에서 v_bus > 부품 등급 상한. 조건이 T_HW 동안 이어지면 브리지를 끄고 래치한다.

persistent since trip
if isempty(trip), since = -1; trip = 0; end
T_HW = prm(2); I_HW = prm(3); VL_HW = prm(4); VS_HW = prm(5); upper = prm(6);
ftype = prm(7); t_f = prm(8); T_GDF = prm(9);
bmode = round(sup(1)); dmode = round(sup(2)); st = round(sup(5));
hb_fault = ftype == 1 && t >= t_f;
dab_fault = ftype == 2 && t >= t_f;
ip = meas(1); ih = meas(2); vl = meas(3); vs = meas(4); vb = meas(5);
if trip < 0.5 && ~hb_fault && bmode ~= 2
    normal = st >= 1 && st <= 5;
    cond = abs(ip) > I_HW || abs(ih) > I_HW || vl > VL_HW || abs(vs) > VS_HW || (normal && vb > upper);
    if cond
        if since < 0, since = t; end
        if t - since >= T_HW - 1e-15, trip = 1; end
    else
        since = -1;
    end
end
gb = [g(:); 0; 0];
if trip > 0.5 || hb_fault || bmode == 2
    gb(1:4) = 0;
elseif bmode == 1
    gb(1:4) = [0; 1; 0; 1];                       % 영벡터: H-브리지 하측 두 소자
end
if dab_fault || dmode == 2
    gb(5:12) = 0;
end
gb(13) = double(sup(3) > 0.5);
gb(14) = double(sup(4) > 0.5);
fl = [double(hb_fault && t >= t_f + T_GDF); trip];
end

== matlab function TB11_R2_FaultMod_SW/Gate_StageB/DAB_EPS_Map ==
  data: sup input; eps output; meas input; prm input; tD input; tP input; tK input
function eps = prism_dab_eps_map(sup, meas, prm, tD, tP, tK)
%#codegen
%PRISM_DAB_EPS_MAP  H-브리지 고장 강등 중 DAB 고장 모드 변조(EPS) 지령(TB10, 검증 코드 E20과 같은 표).
%
%  강등 상태(9 유지, 10 링크 붕괴, 11 소프트 투입)에서 DAB 모드가 보조 지령(1)이면, 상태기계의 보조 링크전류 지령을
%  1차 내부 위상천이(EPS) 지령 [등가 위상 φ; 내부 위상비 D1]로 바꾼다. 게이트 생성기(ctrl/prism_gate_stageB_e.m)는
%  1차 두 레그 가운데 레그 2를 D1·T/2만큼 늦춰 1차 전압에 영구간을 넣고, 2차는 φ만큼 위상을 둔 구형파로 둔다.
%
%  정규화(2차 환산): V1' = v_bus/n, ωL' = 2π f_s L_dab/n², I_b = V1'/ωL', r = v_link/V1', j = 지령/I_b.
%  표(검증 코드 dab_modulation.py가 만든 것을 TB10_init.m이 읽음): r(행) × j(열, −0.78–0, 링크 → 1차만)마다
%    tD 1차 펄스 폭 d [rad](D1 = 1 − d/π), tP 등가 위상 φ [rad], tK 정규화 첨두.
%  첨두 상한: 같은 r에서 tK ≤ pk_max/I_b인 가장 큰 |j|까지만 지령한다(나머지 링크전력은 제동 저항이 받음).
%  링크를 채우는 지령(j > 0)은 내지 않는다(강등 중 링크는 다이오드 정류 전류로 채워진다).
%
%  입력  sup   상태기계 지령 12개(5 DAB 모드, 6 보조 링크전류 지령, 11 상태)
%        meas  [v_bus v_link]
%        prm   [켬 n L_dab f_s pk_max r0 dr j0 dj]
%  출력  eps   [EPS 켬; φ; D1]

on = prm(1) > 0.5 && round(sup(5)) == 1 && round(sup(11)) >= 9 && round(sup(11)) <= 11;
eps = [0; 0; 0];
if ~on
    return
end
n = prm(2); Ld = prm(3); fs = prm(4); pkmax = prm(5);
r0 = prm(6); dr = prm(7); j0 = prm(8); dj = prm(9);
[nr, nj] = size(tD);
v1 = max(meas(1), 1)/n;
Ib = v1/(2*pi*fs*Ld/(n*n));
r = min(max(meas(2)/v1, r0), r0 + (nr - 1)*dr);
ir = min(floor((r - r0)/dr) + 1, nr - 1); fr = (r - r0)/dr - (ir - 1);
% 첨두 상한을 지키는 최대 |j|(j = 0 열에서 음의 방향으로)
tgt = pkmax/Ib;
jl = 0;
for k = nj:-1:1
    pk = (1 - fr)*tK(ir, k) + fr*tK(ir + 1, k);
    if pk > tgt
        break
    end
    jl = -(j0 + (k - 1)*dj);
end
jn = min(max(sup(6)/Ib, -jl), 0);
jn = max(jn, j0);
ij = min(floor((jn - j0)/dj) + 1, nj - 1); fj = (jn - j0)/dj - (ij - 1);
d  = (1 - fr)*(1 - fj)*tD(ir, ij) + (1 - fr)*fj*tD(ir, ij + 1) + fr*(1 - fj)*tD(ir + 1, ij) + fr*fj*tD(ir + 1, ij + 1);
ph = (1 - fr)*(1 - fj)*tP(ir, ij) + (1 - fr)*fj*tP(ir, ij + 1) + fr*(1 - fj)*tP(ir + 1, ij) + fr*fj*tP(ir + 1, ij + 1);
D1 = min(max(1 - d/pi, 0), 0.95);
eps = [1; ph; D1];
end
